simulink model "all_cc_0001_0026"  (R2026a)
settings: Solver=VariableStepAuto  StartTime=0  StopTime=100  FixedStep=0.1  MinStep=0.01  AbsTol=1e-5  EnableMultiTasking=on
settings Model: Creator=yoriyuki  LastModifiedBy=harry_31916
settings DataIOCC: ExternalInput=[Throttle, Brake]  FinalStateName=SavePoint  InitialState=SavePoint  SaveOperatingPoint=on  StateSaveName=x  TimeSaveName=t  OutputSaveName=y

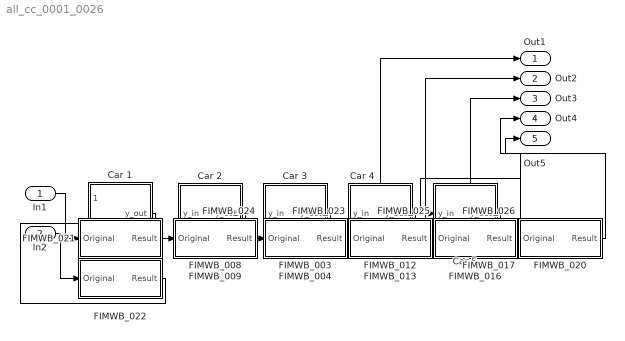
== system all_cc_0001_0026 ==
  In1 : Inport
  In2 : Inport  Port=2
  Car 1 : Stateflow chart  TreatAsAtomicUnit=on
  Car 2 : Stateflow chart  TreatAsAtomicUnit=on
  Car 3 : Stateflow chart  TreatAsAtomicUnit=on
  Car 4 : Stateflow chart  TreatAsAtomicUnit=on
  Car 5 : Stateflow chart  TreatAsAtomicUnit=on
  FIMWB_003 : Subsystem  Tag=fimwb.fault.3
  FIMWB_004 : Subsystem  Tag=fimwb.fault.4
  FIMWB_008 : Subsystem  Tag=fimwb.fault.8
  FIMWB_009 : Subsystem  Tag=fimwb.fault.9
  FIMWB_012 : Subsystem  Tag=fimwb.fault.12
  FIMWB_013 : Subsystem  Tag=fimwb.fault.13
  FIMWB_016 : Subsystem  Tag=fimwb.fault.16
  FIMWB_017 : Subsystem  Tag=fimwb.fault.17
  FIMWB_020 : Subsystem  Tag=fimwb.fault.20
  FIMWB_021 : Subsystem  Tag=fimwb.fault.21
  FIMWB_022 : Subsystem  Tag=fimwb.fault.22
  FIMWB_023 : Subsystem  Tag=fimwb.fault.23
  FIMWB_024 : Subsystem  Tag=fimwb.fault.24
  FIMWB_025 : Subsystem  Tag=fimwb.fault.25
  FIMWB_026 : Subsystem  Tag=fimwb.fault.26
  Out1 : Outport  VectorParamsAs1DForOutWhenUnconnected=off
  Out2 : Outport  Port=2  VectorParamsAs1DForOutWhenUnconnected=off
  Out3 : Outport  Port=3  VectorParamsAs1DForOutWhenUnconnected=off
  Out4 : Outport  Port=4  VectorParamsAs1DForOutWhenUnconnected=off
  Out5 : Outport  Port=5  VectorParamsAs1DForOutWhenUnconnected=off
  wires:
  Car 2/1(y_out) -> FIMWB_023/1(Original)
  FIMWB_023/1(Result) -> FIMWB_003/1(Original), FIMWB_004/1(Original)
  Car 1/1(y_out) -> FIMWB_024/1(Original)
  FIMWB_024/1(Result) -> FIMWB_008/1(Original), FIMWB_009/1(Original)
  Car 3/1(y_out) -> FIMWB_025/1(Original)
  FIMWB_025/1(Result) -> FIMWB_012/1(Original), FIMWB_013/1(Original)
  Car 4/1(y_out) -> FIMWB_026/1(Original)
  FIMWB_026/1(Result) -> FIMWB_016/1(Original), FIMWB_017/1(Original)
  FIMWB_003/1(Result) -> Car 3/1(y_in)
  FIMWB_004/1(Result) -> Out2/1
  FIMWB_008/1(Result) -> Car 2/1(y_in)
  FIMWB_009/1(Result) -> Out1/1
  FIMWB_012/1(Result) -> Car 4/1(y_in)
  FIMWB_013/1(Result) -> Out3/1
  FIMWB_016/1(Result) -> Car 5/1(y_in)
  FIMWB_017/1(Result) -> Out4/1
  Car 5/1(y_out) -> FIMWB_020/1(Original)
  FIMWB_020/1(Result) -> Out5/1
  In1/1 -> FIMWB_021/1(Original)
  FIMWB_021/1(Result) -> Car 1/1(Throttle)
  In2/1 -> FIMWB_022/1(Original)
  FIMWB_022/1(Result) -> Car 1/2(Brake)

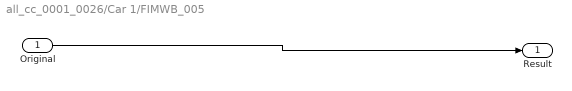
== system all_cc_0001_0026/Car 1/FIMWB_005 ==
  Original : Inport
  Result : Outport
  wires:
  Original/1 -> Result/1

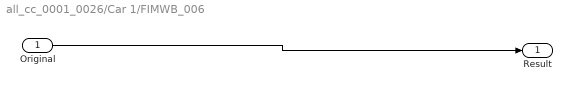
== system all_cc_0001_0026/Car 1/FIMWB_006 ==
  Original : Inport
  Result : Outport
  wires:
  Original/1 -> Result/1

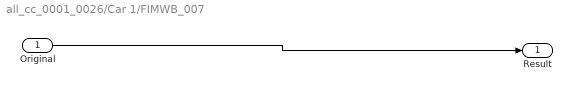
== system all_cc_0001_0026/Car 1/FIMWB_007 ==
  Original : Inport
  Result : Outport
  wires:
  Original/1 -> Result/1

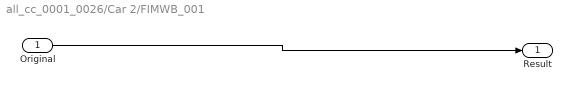
== system all_cc_0001_0026/Car 2/FIMWB_001 ==
  Original : Inport
  Result : Outport
  wires:
  Original/1 -> Result/1

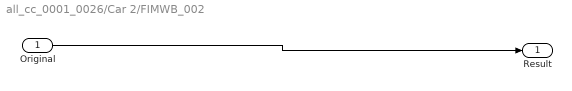
== system all_cc_0001_0026/Car 2/FIMWB_002 ==
  Original : Inport
  Result : Outport
  wires:
  Original/1 -> Result/1

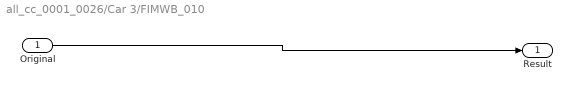
== system all_cc_0001_0026/Car 3/FIMWB_010 ==
  Original : Inport
  Result : Outport
  wires:
  Original/1 -> Result/1

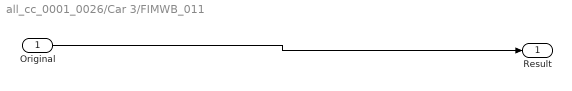
== system all_cc_0001_0026/Car 3/FIMWB_011 ==
  Original : Inport
  Result : Outport
  wires:
  Original/1 -> Result/1

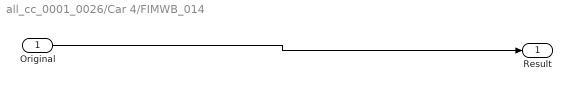
== system all_cc_0001_0026/Car 4/FIMWB_014 ==
  Original : Inport
  Result : Outport
  wires:
  Original/1 -> Result/1

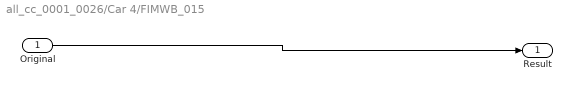
== system all_cc_0001_0026/Car 4/FIMWB_015 ==
  Original : Inport
  Result : Outport
  wires:
  Original/1 -> Result/1

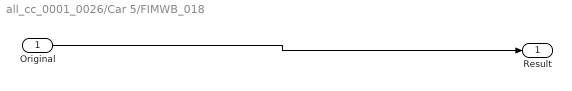
== system all_cc_0001_0026/Car 5/FIMWB_018 ==
  Original : Inport
  Result : Outport
  wires:
  Original/1 -> Result/1

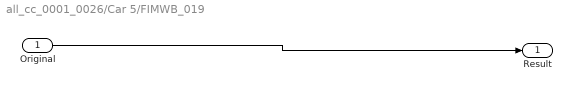
== system all_cc_0001_0026/Car 5/FIMWB_019 ==
  Original : Inport
  Result : Outport
  wires:
  Original/1 -> Result/1

== system all_cc_0001_0026/FIMWB_003 ==
  Original : Inport
  Result : Outport
  wires:
  Original/1 -> Result/1

== system all_cc_0001_0026/FIMWB_004 ==
  Original : Inport
  Result : Outport
  wires:
  Original/1 -> Result/1

== system all_cc_0001_0026/FIMWB_008 ==
  Original : Inport
  Result : Outport
  wires:
  Original/1 -> Result/1

== system all_cc_0001_0026/FIMWB_009 ==
  Original : Inport
  Result : Outport
  wires:
  Original/1 -> Result/1

== system all_cc_0001_0026/FIMWB_012 ==
  Original : Inport
  Result : Outport
  wires:
  Original/1 -> Result/1

== system all_cc_0001_0026/FIMWB_013 ==
  Original : Inport
  Result : Outport
  wires:
  Original/1 -> Result/1

== system all_cc_0001_0026/FIMWB_016 ==
  Original : Inport
  Result : Outport
  wires:
  Original/1 -> Result/1

== system all_cc_0001_0026/FIMWB_017 ==
  Original : Inport
  Result : Outport
  wires:
  Original/1 -> Result/1

== system all_cc_0001_0026/FIMWB_020 ==
  Original : Inport
  Result : Outport
  wires:
  Original/1 -> Result/1

== system all_cc_0001_0026/FIMWB_021 ==
  Original : Inport
  Result : Outport
  wires:
  Original/1 -> Result/1

== system all_cc_0001_0026/FIMWB_022 ==
  Original : Inport
  Result : Outport
  wires:
  Original/1 -> Result/1

== system all_cc_0001_0026/FIMWB_023 ==
  Original : Inport
  Result : Outport
  wires:
  Original/1 -> Result/1

== system all_cc_0001_0026/FIMWB_024 ==
  Original : Inport
  Result : Outport
  wires:
  Original/1 -> Result/1

== system all_cc_0001_0026/FIMWB_025 ==
  Original : Inport
  Result : Outport
  wires:
  Original/1 -> Result/1

== system all_cc_0001_0026/FIMWB_026 ==
  Original : Inport
  Result : Outport
  wires:
  Original/1 -> Result/1

== stateflow chart all_cc_0001_0026/Car 1 ==
  settings: updateMethod=CONTINUOUS
  state Run
    during:
    v_dot = -Throttle - Brake * v;
    y_dot = v;
    y_out = y;
  (default) -> Run
  data: Throttle input; Brake input; y local =0; y_out output; v local =0
  data y settings: updateMethod=SF_CONTINUOUS_TIME_DATA
  data v settings: updateMethod=SF_CONTINUOUS_TIME_DATA

== stateflow chart all_cc_0001_0026/Car 3 ==
  settings: updateMethod=CONTINUOUS
  state Chasing
    during:
    v_dot = 1;
    y_dot = -v;
    y_out = y;
  state Keeping
    during:
    y_dot = v;
    y_out = y;
  state Braking
    during:
    v_dot = -v;
    y_dot = -v;
    y_out = y;
  (default) -> Keeping
  Chasing -> Keeping : [y - y_in <= 10]
      | % [transition condition]{action}
  Keeping -> Chasing [order 1] : [y - y_in >=15]
  Braking -> Chasing : [y - y_in >= 20]
  Keeping -> Braking [order 2] : [y - y_in <=5]
  data: y_out output; y local double =20; v local =0; y_in input
  data y settings: updateMethod=SF_CONTINUOUS_TIME_DATA
  data v settings: updateMethod=SF_CONTINUOUS_TIME_DATA
  data y_in settings: updateMethod=SF_CONTINUOUS_TIME_DATA

== stateflow chart all_cc_0001_0026/Car 2 ==
  settings: updateMethod=CONTINUOUS
  state Chasing
    during:
    v_dot = 1;
    y_dot = -v;
    y_out = y;
  state Keeping
    during:
    y_dot = v;
    y_out = y;
  state Braking
    during:
    v_dot = -v;
    y_dot = -v;
    y_out = y;
  (default) -> Keeping
  Chasing -> Keeping : [y - y_in <= 10]
  Keeping -> Chasing [order 1] : [y - y_in >=15]
  Braking -> Chasing : [y - y_in >= 20]
  Keeping -> Braking [order 2] : [y - y_in <=5]
  data: y_out output; y local double =10; v local =0; y_in input
  data y settings: updateMethod=SF_CONTINUOUS_TIME_DATA
  data v settings: updateMethod=SF_CONTINUOUS_TIME_DATA
  data y_in settings: updateMethod=SF_CONTINUOUS_TIME_DATA

== stateflow chart all_cc_0001_0026/Car 4 ==
  settings: updateMethod=CONTINUOUS
  state Chasing
    during:
    v_dot = 1;
    y_dot = -v;
    y_out = y;
  state Keeping
    during:
    y_dot = v;
    y_out = y;
  state Braking
    during:
    v_dot = -v;
    y_dot = -v;
    y_out = y;
  (default) -> Keeping
  Chasing -> Keeping : [y - y_in <= 10]
      | % [transition condition]{action}
  Keeping -> Chasing [order 1] : [y - y_in >=15]
  Braking -> Chasing : [y - y_in >= 20]
  Keeping -> Braking [order 2] : [y - y_in <=5]
  data: y local double =30; v local =0; y_in input; y_out output
  data y settings: updateMethod=SF_CONTINUOUS_TIME_DATA
  data v settings: updateMethod=SF_CONTINUOUS_TIME_DATA
  data y_in settings: updateMethod=SF_CONTINUOUS_TIME_DATA

== stateflow chart all_cc_0001_0026/Car 5 ==
  settings: updateMethod=CONTINUOUS
  state Keeping
    during:
    y_dot = v;
    y_out = y;
  state Chasing
    during:
    v_dot = 1;
    y_dot = -v;
    y_out = y;
  state Braking
    during:
    v_dot = -v;
    y_dot = -v;
    y_out = y;
  (default) -> Keeping
  Chasing -> Keeping : [y - y_in <= 10]
      | % [transition condition]{action}
  Keeping -> Chasing [order 1] : [y - y_in >=15]
  Braking -> Chasing : [y - y_in >= 20]
  Keeping -> Braking [order 2] : [y - y_in <=5]
  data: y_out output; y local double =40; v local =0; y_in input
  data y settings: updateMethod=SF_CONTINUOUS_TIME_DATA
  data v settings: updateMethod=SF_CONTINUOUS_TIME_DATA
  data y_in settings: updateMethod=SF_CONTINUOUS_TIME_DATA
